simulink model "therm"  (R2024a)
settings: Solver=VariableStepAuto  StartTime=0.0  StopTime=inf  RelTol=1e-3
values from neighbouring files (symbols this model uses):
  Iin = Iin_array(i)    [peltierscript.m]
  Tcold = Tcold_array(j)    [peltierscript.m]
undefined symbols (not defined in the file or in its folder): tol
libraries: fl_lib x14, nesl_utility x8, simulink x1, ee_lib x1
settings Model: Creator=THEOFANIDIS  LastModifiedBy=Theof
settings DebuggingCC: UnconnectedInputMsg=warning  UnconnectedOutputMsg=warning  UnconnectedLineMsg=warning
settings ModelReferenceCC: EnableRefExpFcnMdlSchedulingChecks=on
settings RTWCC: GPUComputeCapability=3.5  DLArmComputeVersion=19.05

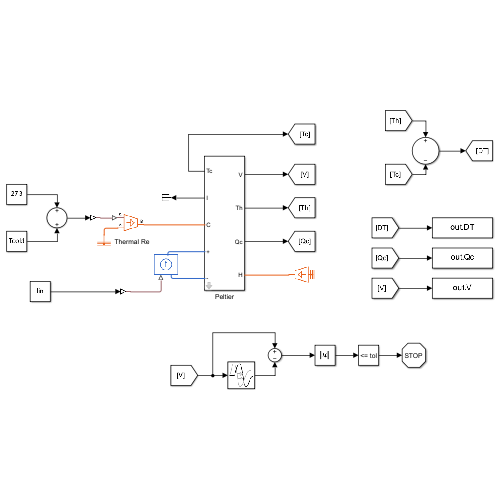
[thumbnail: Simulink's stored preview of the top-level diagram]
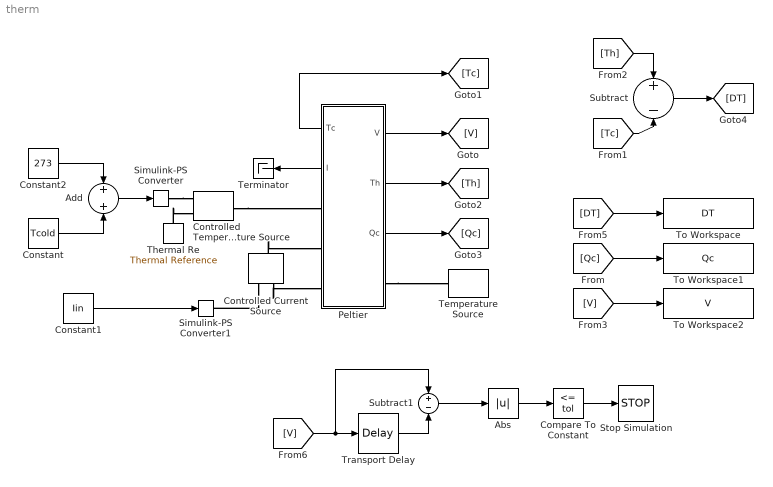
== system therm ==
  Abs : Abs  SaturateOnIntegerOverflow=off
  Add : Sum
  Compare To Constant : simulink/Logic and Bit Operations/Compare To Constant  relop=<=  const=tol  OutDataTypeStr=boolean
  Constant : Constant  Value=Tcold
  Constant1 : Constant  Value=Iin
  Constant2 : Constant  Value=273
  Controlled Temperature Source : fl_lib/Thermal/Thermal Sources/Controlled Temperature Source
  Controlled Current Source : fl_lib/Electrical/Electrical Sources/Controlled Current Source
  Peltier : Subsystem  mask{S=0.053, R=2, Rth=2, Cth=20}
      mask prompts: S "Seebeck coeff"; R "Resistance"; Rth "Thermal Resistance"; Cth "Thermal Capacity"
      settings: PortSchema="{\"entries\":[{\"content\":{\"sides\":[{\"content\":{\"connectorIds\":[\"Out4\",\"Out5\",\"LConn1\",\"LConn2\",\"LConn3\"]},\"type\":\"ConnectorPlacement.EquallySpacedRectSide\",\"uuid\":\"7b612d58-64a3-456b-8c94-0b47eb8aef96\"},{\"content\":{\"connectorIds\":[\"Out1\",\"Out2\",\"Out3\",\"RConn1\"],\"side\":\"RIGHT\"},\"type\":\"ConnectorPlacement.EquallySpacedRectSide\",\"uuid\":\"2f2d1fc6-4c28-432f-83e8-52c7cae39343\"},{\"content\":{\"connectorIds\":[],\"side\":\"TOP\"},\"type\":\"ConnectorPlacement.EquallySpacedRectSide\",\"uuid\":\"b65206c2-8afd-44bb-a455-6ebd5e3b3815\"}]},\"type\":\"ConnectorPlacement.EquallySpacedConnector\",\"uuid\":\"72c1d7be-9b5b-4c47-b998-86198d006e1c\"}],\"packageUris\":[\"http://schema.mathworks.com/mf0/Connector/R2020b\"],\"version\":\"1.0\"}"
  Simulink-PS Converter : nesl_utility/Simulink-PS Converter  PhysicalDomain=network_engine_domain  SubClassName=ps_input  LeftPortType=input  RightPortType=output  PseudoPeriodic=off  Frequencies=[]  NoiseDistribution=none  NoiseParameters=[]  Unit=1  AffineConversion=off  FilteringAndDerivatives=provide  SimscapeFilterOrder=1  InputFilterTimeConstant=0.001  UdotUserProvided=0
  Simulink-PS Converter1 : nesl_utility/Simulink-PS Converter  PhysicalDomain=network_engine_domain  SubClassName=ps_input  LeftPortType=input  RightPortType=output  PseudoPeriodic=off  Frequencies=[]  NoiseDistribution=none  NoiseParameters=[]  Unit=1  AffineConversion=off  FilteringAndDerivatives=provide  SimscapeFilterOrder=1  InputFilterTimeConstant=0.001  UdotUserProvided=0
  Stop Simulation : Stop
  Subtract : Sum  Inputs=+-
  Subtract1 : Sum  Inputs=+-
  Temperature Source : fl_lib/Thermal/Thermal Sources/Temperature Source  temperature=50 degC
  Terminator : Terminator
  Thermal Re : fl_lib/Thermal/Thermal Elements/Thermal Reference
  To Workspace : ToWorkspace  VariableName=DT  SampleTime=-1
  To Workspace1 : ToWorkspace  VariableName=Qc  SampleTime=-1
  To Workspace2 : ToWorkspace  VariableName=V  SampleTime=-1
  Transport Delay : TransportDelay
  wires:
  Peltier/1(V) -> [V]
  Peltier/4(Tc) -> [Tc]
  Peltier/2(Th) -> [Th]
  Peltier/3(Qc) -> [Qc]
  [Th] -> Subtract/1
  [Tc] -> Subtract/2
  Subtract/1 -> [DT]
  [DT] -> To Workspace/1
  [Qc] -> To Workspace1/1
  [V] -> To Workspace2/1
  Constant/1 -> Add/2
  Constant2/1 -> Add/1
  Add/1 -> Simulink-PS Converter/1
  [V] -> Transport Delay/1, Subtract1/1
  Transport Delay/1 -> Subtract1/2
  Subtract1/1 -> Abs/1
  Abs/1 -> Compare To Constant/1
  Compare To Constant/1 -> Stop Simulation/1
  Constant1/1 -> Simulink-PS Converter1/1
  Peltier/5(I) -> Terminator/1
  connections:
  Peltier/RConn1 -- Temperature Source/LConn1
  Controlled Temperature Source/LConn1 -- Peltier/LConn1
  Thermal Re/LConn1 -- Controlled Temperature Source/RConn2
  Simulink-PS Converter/RConn1 -- Controlled Temperature Source/RConn1
  Controlled Current Source/RConn1 -- Simulink-PS Converter1/RConn1
  Controlled Current Source/LConn1 -- Peltier/LConn2
  Controlled Current Source/RConn2 -- Peltier/LConn3

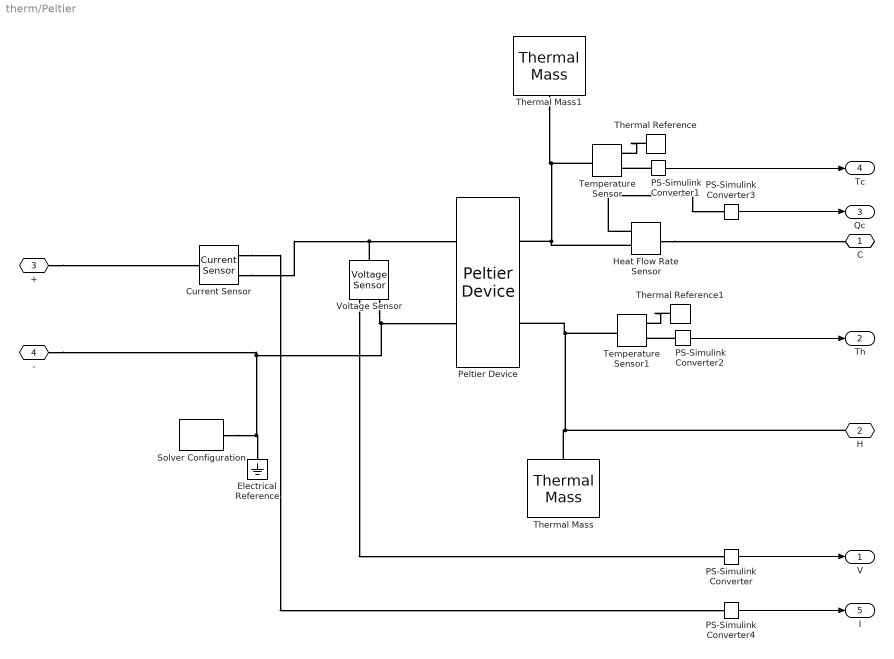
== system therm/Peltier ==
  Current Sensor : fl_lib/Electrical/Electrical Sensors/Current Sensor
  Electrical Reference : fl_lib/Electrical/Electrical Elements/Electrical Reference
  Heat Flow Rate Sensor : fl_lib/Thermal/Thermal Sensors/Heat Flow Rate Sensor
  PS-Simulink Converter{,1..4} (5 alike) : nesl_utility/PS-Simulink Converter  PhysicalDomain=network_engine_domain  SubClassName=ps_output  LeftPortType=input  RightPortType=output  PseudoPeriodic=off  Frequencies=[]  VectorFormat=1-D array  Unit=inherit  AffineConversion=off
  Peltier Device : ee_lib/Sensors & Transducers/Peltier Device  alpha=S V/K  R=R Ohm  K=1/Rth W/K
      settings: InternalSimscapePortConfiguration="{\"Bottom\":[],\"Left\":[{\"id\":\"p\",\"label\":\"+\",\"type\":\"foundation.electrical.electrical\"},{\"id\":\"n\",\"label\":\"-\",\"type\":\"foundation.electrical.electrical\"}],\"Right\":[{\"id\":\"A\",\"label\":\"A\",\"type\":\"foundation.thermal.thermal\"},{\"id\":\"B\",\"label\":\"B\",\"type\":\"foundation.thermal.thermal\"}],\"Top\":[]}"
  Solver Configuration : nesl_utility/Solver Configuration  PhysicalDomain=network_engine_domain  SubClassName=solver  LeftPortType=input  RightPortType=generic  Tones=[]  Harmonics=[]  SimulateNoise=off  Profile=off  UseLocalSampling=off  EnableSwitchedLinearOptims=on  FrequencyDomain=off  UseCCode=off  RelTol=0.001  AbsTol=1e-06  MinStep=1e-09  ToWorkspace=off  RevertToSquareIcSolve=off  NumHomotopyIterations=100  PhasorMode=off  PhasorModeNumHarmonics=1  ConsistencySolver=NEWTON_FTOL  IndexReductionMethod=DerivativeReplacement  DoDC=off  ResidualTolerance=1e-09  ConsistencyTolSource=GLOBAL  ConsistencyAbsTol=0.001  ConsistencyRelTol=0.001  ConsistencyTolFactor=0.001  UseLocalSolver=off  LocalSolverChoice=NE_BACKWARD_EULER_ADVANCER  ResolveIndetEquations=on  FunctionEvalNumThread=1  LocalSolverSampleTime=0.001  DoFixedCost=off  MaxNonlinIter=3  MaxModeIter=2  ComputeImpulses=off  ImpulseIterations=2  LinearAlgebra=auto  LinearAlgebraNumThread=0  EquationFormulation=NE_TIME_EF  DelaysMemoryBudget=1024  AutomaticFiltering=on  FilteringTimeConstant=0.001  PartitionStorageMethod=AS_NEEDED  PartitionMemoryBudget=1024  PartitionMethod=ROBUST  MultibodyUseLocalSolver=off  MultibodyLocalSolverChoice=ODE1  MultibodyLocalSolverSampleTime=0.001
  Temperature Sensor : fl_lib/Thermal/Thermal Sensors/Temperature Sensor  temperature_measure=foundation.enum.MeasurementReference.difference
  Temperature Sensor1 : fl_lib/Thermal/Thermal Sensors/Temperature Sensor  temperature_measure=foundation.enum.MeasurementReference.difference
  Thermal Mass : fl_lib/Thermal/Thermal Elements/Thermal Mass  mass_type=foundation.enum.constant_variable.constant  mass=12 g  sp_heat=Cth/2/0.012 J/(K*kg)  mass_min=1e-6 kg  num_ports=foundation.enum.numPorts2.one  m_specify=off  m_priority=High  m=1 kg  m_nominal_specify=off  m_nominal_value=1  m_nominal_unit=kg  T_specify=off  T_priority=High  T=300 K  T_nominal_specify=off  T_nominal_value=1  T_nominal_unit=K  Q_specify=off  Q_priority=None  Q=0 W  Q_nominal_specify=off  Q_nominal_value=1  Q_nominal_unit=W
  Thermal Mass1 : fl_lib/Thermal/Thermal Elements/Thermal Mass  mass_type=foundation.enum.constant_variable.constant  mass=12 g  sp_heat=Cth/2/0.012 J/(K*kg)  mass_min=1e-6 kg  num_ports=foundation.enum.numPorts2.one  m_specify=off  m_priority=High  m=1 kg  m_nominal_specify=off  m_nominal_value=1  m_nominal_unit=kg  T_specify=off  T_priority=High  T=300 K  T_nominal_specify=off  T_nominal_value=1  T_nominal_unit=K  Q_specify=off  Q_priority=None  Q=0 W  Q_nominal_specify=off  Q_nominal_value=1  Q_nominal_unit=W
  Thermal Reference : fl_lib/Thermal/Thermal Elements/Thermal Reference
  Thermal Reference1 : fl_lib/Thermal/Thermal Elements/Thermal Reference
  Voltage Sensor : fl_lib/Electrical/Electrical Sensors/Voltage Sensor
  C : PMIOPort  Side=Left
  H : PMIOPort  Port=2  Side=Right
  + : PMIOPort  Port=3  Side=Left
  - : PMIOPort  Port=4  Side=Left
  V : Outport
  Th : Outport  Port=2
  Qc : Outport  Port=3
  Tc : Outport  Port=4
  I : Outport  Port=5
  wires:
  PS-Simulink Converter/1 -> V/1
  PS-Simulink Converter3/1 -> Qc/1
  PS-Simulink Converter1/1 -> Tc/1
  PS-Simulink Converter2/1 -> Th/1
  PS-Simulink Converter4/1 -> I/1
  connections:
  Voltage Sensor/RConn1 -- PS-Simulink Converter/LConn1
  Voltage Sensor/LConn1 -- Peltier Device/LConn1 -- Current Sensor/RConn2
  Temperature Sensor/LConn1 -- Thermal Mass1/LConn1 -- Heat Flow Rate Sensor/RConn2 -- Peltier Device/RConn1
  Heat Flow Rate Sensor/RConn1 -- PS-Simulink Converter3/LConn1
  Temperature Sensor1/LConn1 -- H/RConn1 -- Thermal Mass/LConn1 -- Peltier Device/RConn2
  Thermal Reference/LConn1 -- Temperature Sensor/RConn1
  PS-Simulink Converter1/LConn1 -- Temperature Sensor/RConn2
  PS-Simulink Converter2/LConn1 -- Temperature Sensor1/RConn2
  Thermal Reference1/LConn1 -- Temperature Sensor1/RConn1
  Solver Configuration/RConn1 -- Peltier Device/LConn2 -- Voltage Sensor/RConn2 -- -/RConn1 -- Electrical Reference/LConn1
  +/RConn1 -- Current Sensor/LConn1
  Current Sensor/RConn1 -- PS-Simulink Converter4/LConn1
  Heat Flow Rate Sensor/LConn1 -- C/RConn1
